simulink model "task"  (R2025a)
settings: Solver=VariableStepAuto  StartTime=0.0  StopTime=24  RelTol=1e-3
values from neighbouring files (symbols this model uses):
  D = 0.25    [main.m]
  i = round(i)    [main.m]
  J = 209 / (10^6)    (= 0.000209)    [main.m]
  J_prop = rho_v * pi * R^4 * h / 2    (= 0.0118116520667)    [main.m]
  K1 = 0.18    [main.m]
  K2 = 0.032    [main.m]
  km = 25 / 1000    (= 0.025)    [main.m]
  kw = 1 / 382    (= 0.00261780104712)    [main.m]
  L = 0.0565 / 1000    (= 5.65e-05)    [main.m]
  R_m = 0.143    [main.m]
  rho = 1000    [main.m]
libraries: simulink x1
settings Model: Creator=user  LastModifiedBy=user

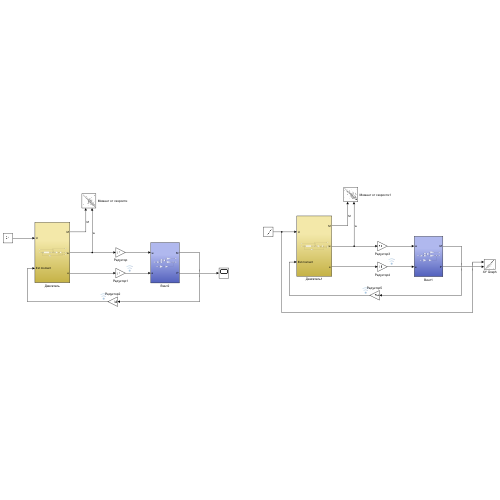
[thumbnail: Simulink's stored preview of the top-level diagram]
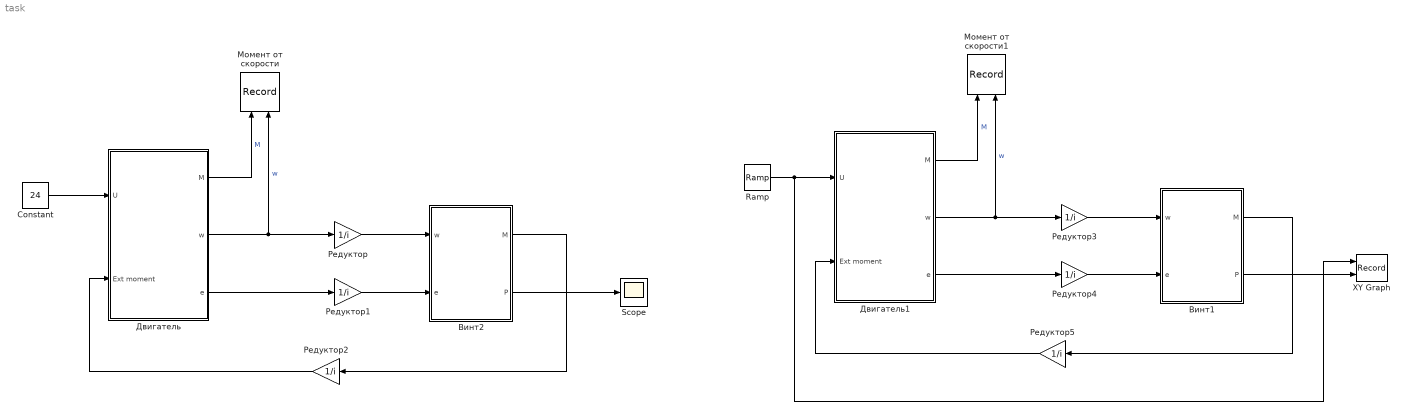
== system task ==
  Constant : Constant  Value=24
  Ramp : simulink/Sources/Ramp  slope=2  start=0  InitialOutput=-24
  Scope : Scope
      settings: ActiveDisplayYMinimum=-8.2863640441226476  ActiveDisplayYMaximum=74.577276397103844
  XY Graph : Record  NumPorts=2.0  FileSettingsInternal="{\"entries\":[{\"content\":{\"excelSettings\":{\"content\":{},\"type\":\"Streamout.ExcelSettings\"},\"parquetSettings\":{\"content\":{},\"type\":\"Streamout.ParquetSettings\"}},\"type\":\"Streamout.FileSettingStorage\",\"uuid\":\"\"}],\"packageUris\":[\"http:\\/\\/schema.mathworks.com\\/mf0\\/streamout_blocks\\/R2020a\"],\"version\":\"1.0\"}"  FrameSettings=[0, 0]  Layout=[1 1]  SignalsInternal="{\"entries\":[{\"content\":{\"signals\":[{\"content\":{\"blockPath\":[],\"dimensions\":[1],\"domain\":\"\",\"lineColor\":\"#a2142f\",\"plots\":[ 1 ],\"port\":1,\"sid\":[\"\"],\"signalID\":1,\"signalName\":\"Ramp\"},\"type\":\"RecordBlkView.Signal\",\"uuid\":\"\"},{\"content\":{\"blockPath\":[],\"dimensions\":[1],\"domain\":\"\",\"lineColor\":\"#139fff\",\"plots\":[ 1 ],\"port\":2,\"sid\":[\"\"],\"signalID\":2,\"signalName\":\"Винт1:2\"},\"type\":\"RecordBlkView.Signal\",\"uuid\":\"\"}]},\"type\":\"RecordBlkView.InputSignals\",\"uuid\":\"\"}],\"packageUris\":[\"http:\\/\\/schema.mathworks.com\\/mf0\\/streamout_blocks\\/R2020a\"],\"version\":\"1.0\"}"  VisualizationBindings="{\"xyplotplugin\":{\"info\":[{\"series\":[{\"bindingParametersList\":[{\"parameter\":\"X-Axis\",\"signalID\":1,\"signalName\":\"Ramp\"},{\"parameter\":\"Y-Axis\",\"signalID\":2,\"signalName\":\"Винт1:2\"}],\"seriesID\":0}],\"subplotID\":1}]}}"  CompatibilityTag=XY
  Винт1 : Subsystem
  Винт2 : Subsystem
  Двигатель : Subsystem
  Двигатель1 : Subsystem
  Момент от скорости : Record  NumPorts=2.0  FileSettingsInternal="{\"entries\":[{\"content\":{\"excelSettings\":{\"content\":{},\"type\":\"Streamout.ExcelSettings\"},\"parquetSettings\":{\"content\":{},\"type\":\"Streamout.ParquetSettings\"}},\"type\":\"Streamout.FileSettingStorage\",\"uuid\":\"\"}],\"packageUris\":[\"http:\\/\\/schema.mathworks.com\\/mf0\\/streamout_blocks\\/R2020a\"],\"version\":\"1.0\"}"  FrameSettings=[0, 0]  Layout=[1 1]  SignalsInternal="{\"entries\":[{\"content\":{\"signals\":[{\"content\":{\"blockPath\":[],\"dimensions\":[1],\"domain\":\"\",\"lineColor\":\"#a2142f\",\"plots\":[ 1 ],\"port\":1,\"sid\":[\"\"],\"signalID\":1,\"signalName\":\"M\"},\"type\":\"RecordBlkView.Signal\",\"uuid\":\"\"},{\"content\":{\"blockPath\":[],\"dimensions\":[1],\"domain\":\"\",\"lineColor\":\"#139fff\",\"plots\":[ 1 ],\"port\":2,\"sid\":[\"\"],\"signalID\":2,\"signalName\":\"w\"},\"type\":\"RecordBlkView.Signal\",\"uuid\":\"\"}]},\"type\":\"RecordBlkView.InputSignals\",\"uuid\":\"\"}],\"packageUris\":[\"http:\\/\\/schema.mathworks.com\\/mf0\\/streamout_blocks\\/R2020a\"],\"version\":\"1.0\"}"  VisualizationBindings="{\"xyplotplugin\":{\"info\":[{\"series\":[{\"bindingParametersList\":[{\"parameter\":\"X-Axis\",\"signalID\":1,\"signalName\":\"M\"},{\"parameter\":\"Y-Axis\",\"signalID\":2,\"signalName\":\"w\"}],\"seriesID\":0}],\"subplotID\":1}]}}"  CompatibilityTag=XY
  Момент от скорости1 : Record  NumPorts=2.0  FileSettingsInternal="{\"entries\":[{\"content\":{\"excelSettings\":{\"content\":{},\"type\":\"Streamout.ExcelSettings\"},\"parquetSettings\":{\"content\":{},\"type\":\"Streamout.ParquetSettings\"}},\"type\":\"Streamout.FileSettingStorage\",\"uuid\":\"\"}],\"packageUris\":[\"http:\\/\\/schema.mathworks.com\\/mf0\\/streamout_blocks\\/R2020a\"],\"version\":\"1.0\"}"  FrameSettings=[0, 0]  Layout=[1 1]  SignalsInternal="{\"entries\":[{\"content\":{\"signals\":[{\"content\":{\"blockPath\":[],\"dimensions\":[1],\"domain\":\"\",\"lineColor\":\"#a2142f\",\"plots\":[ 1 ],\"port\":1,\"sid\":[\"\"],\"signalID\":1,\"signalName\":\"M\"},\"type\":\"RecordBlkView.Signal\",\"uuid\":\"\"},{\"content\":{\"blockPath\":[],\"dimensions\":[1],\"domain\":\"\",\"lineColor\":\"#139fff\",\"plots\":[ 1 ],\"port\":2,\"sid\":[\"\"],\"signalID\":2,\"signalName\":\"w\"},\"type\":\"RecordBlkView.Signal\",\"uuid\":\"\"}]},\"type\":\"RecordBlkView.InputSignals\",\"uuid\":\"\"}],\"packageUris\":[\"http:\\/\\/schema.mathworks.com\\/mf0\\/streamout_blocks\\/R2020a\"],\"version\":\"1.0\"}"  VisualizationBindings="{\"xyplotplugin\":{\"info\":[{\"series\":[{\"bindingParametersList\":[{\"parameter\":\"X-Axis\",\"signalID\":1,\"signalName\":\"M\"},{\"parameter\":\"Y-Axis\",\"signalID\":2,\"signalName\":\"w\"}],\"seriesID\":0}],\"subplotID\":1}]}}"  CompatibilityTag=XY
  Редуктор{,1..5} (6 alike) : Gain  Gain=1/i
  wires:
  Constant/1 -> Двигатель/1(U)
  Двигатель/1(M) -> Момент от скорости/1  "M"
  Двигатель/2(w) -> Момент от скорости/2, Редуктор/1  "w"
  Двигатель/3(e) -> Редуктор1/1
  Редуктор/1 -> Винт2/1(w)
  Редуктор1/1 -> Винт2/2(e)
  Винт2/1(M) -> Редуктор2/1
  Винт2/2(P) -> Scope/1
  Редуктор2/1 -> Двигатель/2(Ext moment)
  Редуктор5/1 -> Двигатель1/2(Ext moment)
  Редуктор4/1 -> Винт1/2(e)
  Винт1/2(P) -> XY Graph/2
  Винт1/1(M) -> Редуктор5/1
  Двигатель1/3(e) -> Редуктор4/1
  Двигатель1/1(M) -> Момент от скорости1/1  "M"
  Двигатель1/2(w) -> Момент от скорости1/2, Редуктор3/1  "w"
  Редуктор3/1 -> Винт1/1(w)
  Ramp/1 -> XY Graph/1, Двигатель1/1(U)

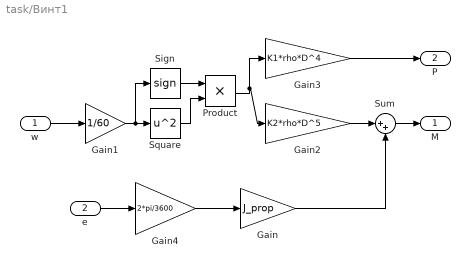
== system task/Винт1 ==
  w : Inport
  e : Inport  Port=2
  Gain : Gain  Gain=J_prop
  Gain1 : Gain  Gain=1/60
  Gain2 : Gain  Gain=K2*rho*D^5
  Gain3 : Gain  Gain=K1*rho*D^4
  Gain4 : Gain  Gain=2*pi/3600
  Product : Product
  Sign : Signum
  Square : Math  Operator=square
  Sum : Sum  Inputs=|++
  M : Outport
  P : Outport  Port=2
  wires:
  w/1 -> Gain1/1
  Gain1/1 -> Sign/1, Square/1
  Square/1 -> Product/2
  Gain2/1 -> Sum/1
  Gain3/1 -> P/1
  e/1 -> Gain4/1
  Gain4/1 -> Gain/1
  Sum/1 -> M/1
  Gain/1 -> Sum/2
  Sign/1 -> Product/1
  Product/1 -> Gain3/1, Gain2/1

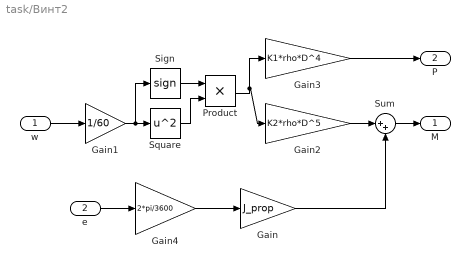
== system task/Винт2 ==
  w : Inport
  e : Inport  Port=2
  Gain : Gain  Gain=J_prop
  Gain1 : Gain  Gain=1/60
  Gain2 : Gain  Gain=K2*rho*D^5
  Gain3 : Gain  Gain=K1*rho*D^4
  Gain4 : Gain  Gain=2*pi/3600
  Product : Product
  Sign : Signum
  Square : Math  Operator=square
  Sum : Sum  Inputs=|++
  M : Outport
  P : Outport  Port=2
  wires:
  w/1 -> Gain1/1
  Gain1/1 -> Sign/1, Square/1
  Square/1 -> Product/2
  Gain2/1 -> Sum/1
  Gain3/1 -> P/1
  e/1 -> Gain4/1
  Gain4/1 -> Gain/1
  Sum/1 -> M/1
  Gain/1 -> Sum/2
  Sign/1 -> Product/1
  Product/1 -> Gain3/1, Gain2/1

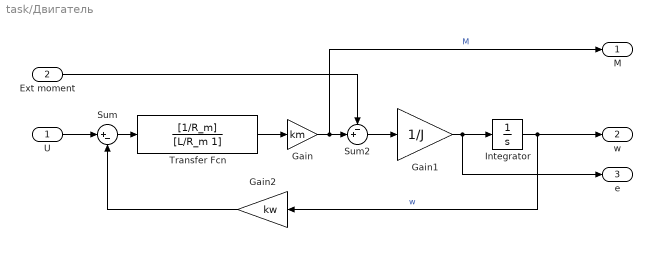
== system task/Двигатель ==
  U : Inport
  Ext moment : Inport  Port=2
  Gain : Gain  Gain=km
  Gain1 : Gain  Gain=1/J
  Gain2 : Gain  Gain=kw
  Integrator : Integrator
  Sum : Sum  Inputs=|+-
  Sum2 : Sum  Inputs=-+|
  Transfer Fcn : TransferFcn  Numerator=[1/R_m]  Denominator=[L/R_m 1]
  M : Outport
  w : Outport  Port=2
  e : Outport  Port=3
  wires:
  Gain1/1 -> e/1, Integrator/1
  Gain/1 -> Sum2/2, M/1  "M"
  Transfer Fcn/1 -> Gain/1
  Integrator/1 -> Gain2/1, w/1  "w"
  Sum/1 -> Transfer Fcn/1
  Gain2/1 -> Sum/2
  U/1 -> Sum/1
  Sum2/1 -> Gain1/1
  Ext moment/1 -> Sum2/1

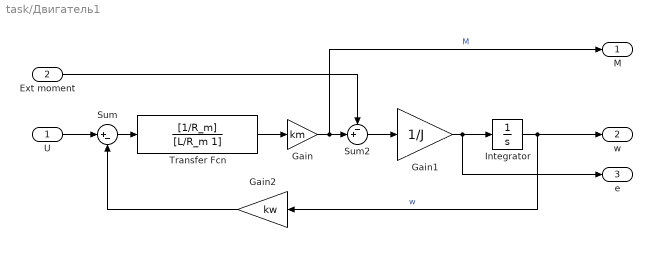
== system task/Двигатель1 ==
  U : Inport
  Ext moment : Inport  Port=2
  Gain : Gain  Gain=km
  Gain1 : Gain  Gain=1/J
  Gain2 : Gain  Gain=kw
  Integrator : Integrator
  Sum : Sum  Inputs=|+-
  Sum2 : Sum  Inputs=-+|
  Transfer Fcn : TransferFcn  Numerator=[1/R_m]  Denominator=[L/R_m 1]
  M : Outport
  w : Outport  Port=2
  e : Outport  Port=3
  wires:
  Gain1/1 -> e/1, Integrator/1
  Gain/1 -> Sum2/2, M/1  "M"
  Transfer Fcn/1 -> Gain/1
  Integrator/1 -> Gain2/1, w/1  "w"
  Sum/1 -> Transfer Fcn/1
  Gain2/1 -> Sum/2
  U/1 -> Sum/1
  Sum2/1 -> Gain1/1
  Ext moment/1 -> Sum2/1
